simulink model "ex2s"  (R2022a)
settings: Solver=VariableStepAuto  StartTime=0.0  StopTime=10.0  MaxStep=0.01  RelTol=1e-3
settings Model: Creator=giova  LastModifiedBy=giova

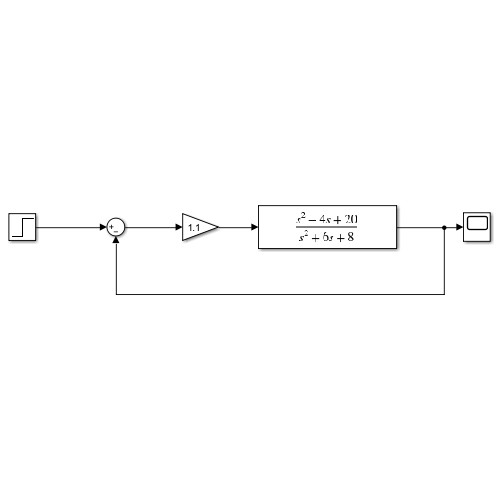
[thumbnail: Simulink's stored preview of the top-level diagram]
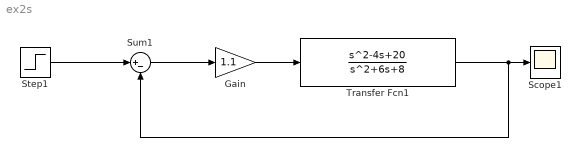
== system ex2s ==
  Gain : Gain  Gain=1.1
  Scope1 : Scope
  Step1 : Step  SampleTime=0
  Sum1 : Sum  Inputs=|+-
  Transfer Fcn1 : TransferFcn  Numerator=[1 -4 20]  Denominator=[1 6 8]
  wires:
  Gain/1 -> Transfer Fcn1/1
  Step1/1 -> Sum1/1
  Sum1/1 -> Gain/1
  Transfer Fcn1/1 -> Sum1/2, Scope1/1
